simulink library "Braccio_lib"  (R2025b)
settings: Solver=VariableStepAuto  StartTime=0.0  StopTime=10.0  RelTol=1e-3
values from neighbouring files (symbols this model uses):
  dt = 0.01    [Braccio_ini.m]    (also in Braccio_kinematics.m)
  eTol = 0.01    [Braccio_ini.m]
  jnt1 = rigidBodyJoint('jnt1','revolute')    [Braccio_ini.m]    (also in Braccio_kinematics.m)
  jnt2 = rigidBodyJoint('jnt2','revolute')    [Braccio_ini.m]    (also in Braccio_kinematics.m)
  jnt3 = rigidBodyJoint('jnt3','revolute')    [Braccio_ini.m]    (also in Braccio_kinematics.m)
  jnt4 = rigidBodyJoint('jnt4','revolute')    [Braccio_ini.m]    (also in Braccio_kinematics.m)
  jnt5 = rigidBodyJoint('jnt5','revolute')    [Braccio_ini.m]    (also in Braccio_kinematics.m)
undefined symbols (not defined in the file or in its folder): cartesianPath, DiscIntNeverNeededParam, jnt6
libraries: simulink x17, robotcorelib x2
settings Model: Creator=Bender  LastModifiedBy=tom

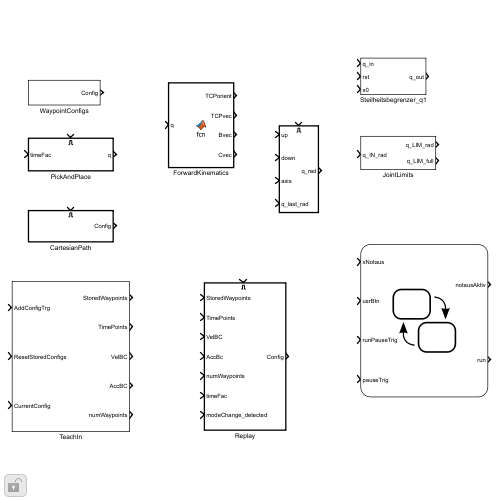
[thumbnail: Simulink's stored preview of the top-level diagram]
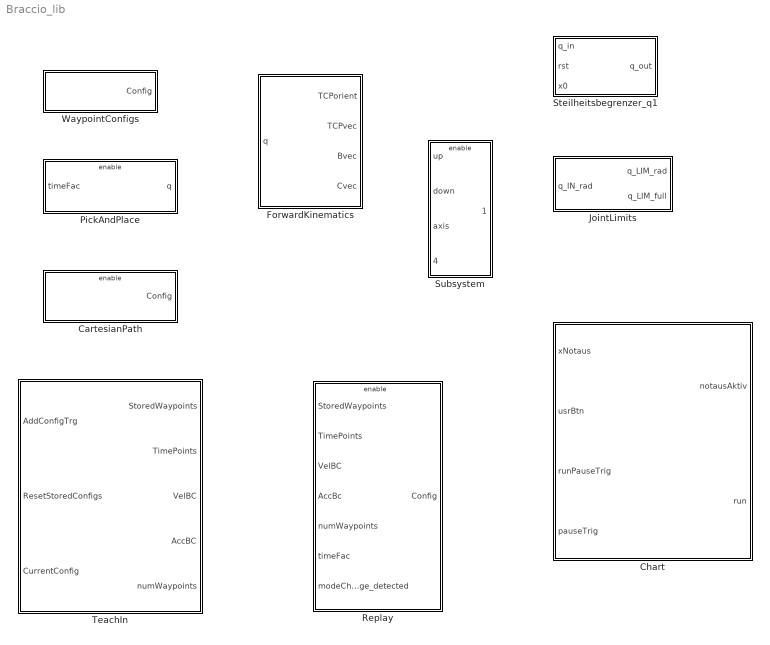
== system Braccio_lib ==
  CartesianPath : Subsystem
  Chart : Stateflow chart  TreatAsAtomicUnit=on
  ForwardKinematics : MATLAB Function  TreatAsAtomicUnit=on
  JointLimits : Subsystem
  PickAndPlace : Subsystem
  Replay : Subsystem
  Steilheitsbegrenzer_q1 : Subsystem
  Subsystem : Subsystem
  TeachIn : Subsystem
  WaypointConfigs : Subsystem

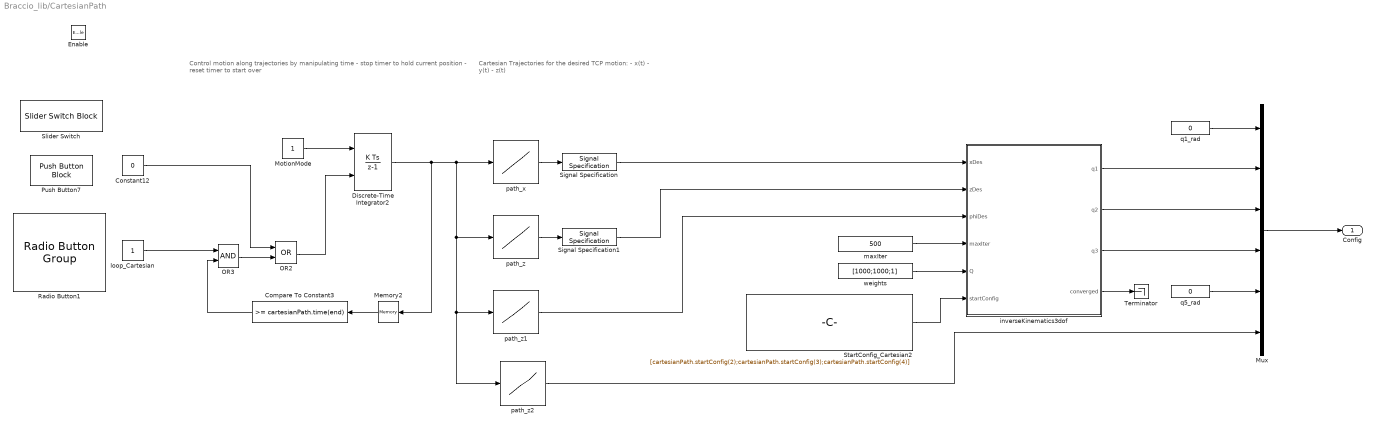
== system Braccio_lib/CartesianPath ==
  note: Cartesian Trajectories for the desired
      | TCP motion:
      | - x(t)
      | - y(t)
      | - z(t)
  note: Control motion along trajectories by manipulating time
      | - stop timer to hold current position
      | - reset timer to start over
  Enable : EnablePort
  Compare To Constant3 : simulink/Logic and Bit Operations/Compare To Constant  relop=>=  const=cartesianPath.time(end)  OutDataTypeStr=boolean
  Constant12 : Constant  Value=0  SampleTime=dt
  Discrete-Time Integrator2 : DiscreteIntegrator  ExternalReset=level  SampleTime=-1  ICPrevOutput=DiscIntNeverNeededParam  ICPrevScaledInput=DiscIntNeverNeededParam
  Memory2 : Memory  InheritSampleTime=on
  MotionMode : Constant  SampleTime=dt
  Mux : Mux  Inputs=6
  OR2 : Logic  Operator=OR  AllPortsSameDT=off  OutDataTypeStr=boolean
  OR3 : Logic  AllPortsSameDT=off  OutDataTypeStr=boolean
  Push Button7 : PushButtonBlock  ButtonText=Reset Time  ButtonType=Latch  IconOnColor=[0.0, 0.39215686274509803, 0.0]  IconOffColor=[0.0, 1.0, 0.0]  OffValue=0.000000
  Radio Button1 : RadioButtonGroup  SelectedLabel=Loop ON  ButtonGroupName=Group
  Signal Specification : SignalSpecification  Dimensions=1
  Signal Specification1 : SignalSpecification  Dimensions=1
  Slider Switch : SliderSwitchBlock
  StartConfig_Cartesian2 : Constant  Value=[cartesianPath.startConfig(2);cartesianPath.startConfig(3);cartesianPath.startConfig(4)]  VectorParams1D=off
  Terminator : Terminator
  inverseKinematics3dof : MATLAB Function  TreatAsAtomicUnit=on
  loop_Cartesian : Constant  SampleTime=dt
  maxIter : Constant  Value=500  SampleTime=dt
  path_x : Lookup_n-D  NumberOfTableDimensions=1  BreakpointsForDimension1=cartesianPath.time  BreakpointsForDimension1DataTypeStr=double  Table=cartesianPath.x  TableDataTypeStr=double  ExtrapMethod=Clip  UseLastTableValue=on  InternalRulePriority=Speed  OutDataTypeStr=double  RndMeth=Simplest
  path_z : Lookup_n-D  NumberOfTableDimensions=1  BreakpointsForDimension1=cartesianPath.time  BreakpointsForDimension1DataTypeStr=double  Table=cartesianPath.z  TableDataTypeStr=double  ExtrapMethod=Clip  UseLastTableValue=on  InternalRulePriority=Speed  OutDataTypeStr=double  RndMeth=Simplest
  path_z1 : Lookup_n-D  NumberOfTableDimensions=1  BreakpointsForDimension1=cartesianPath.time  BreakpointsForDimension1DataTypeStr=double  Table=cartesianPath.angle  TableDataTypeStr=double  ExtrapMethod=Clip  UseLastTableValue=on  InternalRulePriority=Speed  OutDataTypeStr=double  RndMeth=Simplest
  path_z2 : Lookup_n-D  NumberOfTableDimensions=1  BreakpointsForDimension1=cartesianPath.time  BreakpointsForDimension1DataTypeStr=double  Table=cartesianPath.q6  TableDataTypeStr=double  ExtrapMethod=Clip  UseLastTableValue=on  InternalRulePriority=Speed  OutDataTypeStr=double  RndMeth=Simplest
  q1_rad : Constant  Value=0  SampleTime=dt
  q5_rad : Constant  Value=0  SampleTime=dt
  weights : Constant  Value=[1000;1000;1]  VectorParams1D=off  SampleTime=dt
  Config : Outport
  wires:
  Constant12/1 -> OR2/1
  loop_Cartesian/1 -> OR3/1
  OR3/1 -> OR2/2
  Discrete-Time Integrator2/1 -> Memory2/1, path_z2/1, path_z1/1, path_z/1, path_x/1
  OR2/1 -> Discrete-Time Integrator2/2
  Memory2/1 -> Compare To Constant3/1
  Compare To Constant3/1 -> OR3/2
  MotionMode/1 -> Discrete-Time Integrator2/1
  path_x/1 -> Signal Specification/1
  path_z/1 -> Signal Specification1/1
  q1_rad/1 -> Mux/1
  inverseKinematics3dof/1(q1) -> Mux/2
  inverseKinematics3dof/2(q2) -> Mux/3
  inverseKinematics3dof/3(q3) -> Mux/4
  q5_rad/1 -> Mux/5
  path_z2/1 -> Mux/6
  maxIter/1 -> inverseKinematics3dof/4(maxIter)
  weights/1 -> inverseKinematics3dof/5(Q)
  path_z1/1 -> inverseKinematics3dof/3(phiDes)
  Mux/1 -> Config/1
  StartConfig_Cartesian2/1 -> inverseKinematics3dof/6(startConfig)
  inverseKinematics3dof/4(converged) -> Terminator/1
  Signal Specification/1 -> inverseKinematics3dof/1(xDes)
  Signal Specification1/1 -> inverseKinematics3dof/2(zDes)

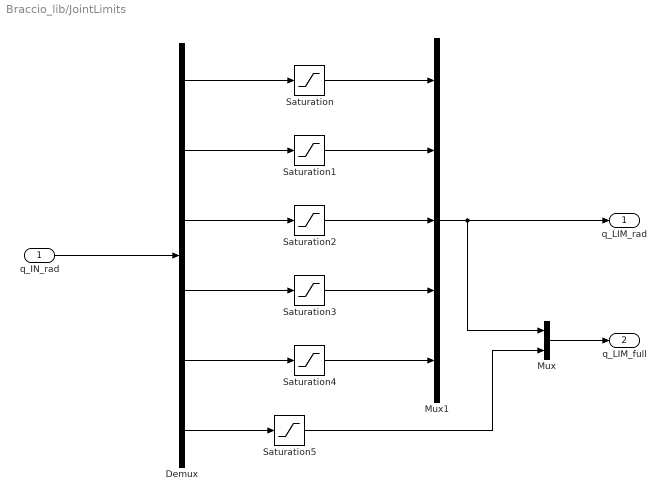
== system Braccio_lib/JointLimits ==
  q_IN_rad : Inport
  Demux : Demux  Outputs=6
  Mux : Mux  Inputs=2
  Mux1 : Mux  Inputs=5
  Saturation : Saturate  UpperLimit=jnt1.PositionLimits(2)  LowerLimit=jnt1.PositionLimits(1)
  Saturation1 : Saturate  UpperLimit=jnt2.PositionLimits(2)  LowerLimit=jnt2.PositionLimits(1)
  Saturation2 : Saturate  UpperLimit=jnt3.PositionLimits(2)  LowerLimit=jnt3.PositionLimits(1)
  Saturation3 : Saturate  UpperLimit=jnt4.PositionLimits(2)  LowerLimit=jnt4.PositionLimits(1)
  Saturation4 : Saturate  UpperLimit=jnt5.PositionLimits(2)  LowerLimit=jnt5.PositionLimits(1)
  Saturation5 : Saturate  UpperLimit=jnt6.PositionLimits(2)  LowerLimit=jnt6.PositionLimits(1)
  q_LIM_rad : Outport
  q_LIM_full : Outport  Port=2
  wires:
  Saturation2/1 -> Mux1/3
  Saturation/1 -> Mux1/1
  Saturation4/1 -> Mux1/5
  Saturation1/1 -> Mux1/2
  Saturation3/1 -> Mux1/4
  Mux1/1 -> Mux/1, q_LIM_rad/1
  q_IN_rad/1 -> Demux/1
  Saturation5/1 -> Mux/2
  Demux/1 -> Saturation/1
  Demux/6 -> Saturation5/1
  Demux/2 -> Saturation1/1
  Demux/3 -> Saturation2/1
  Demux/4 -> Saturation3/1
  Demux/5 -> Saturation4/1
  Mux/1 -> q_LIM_full/1

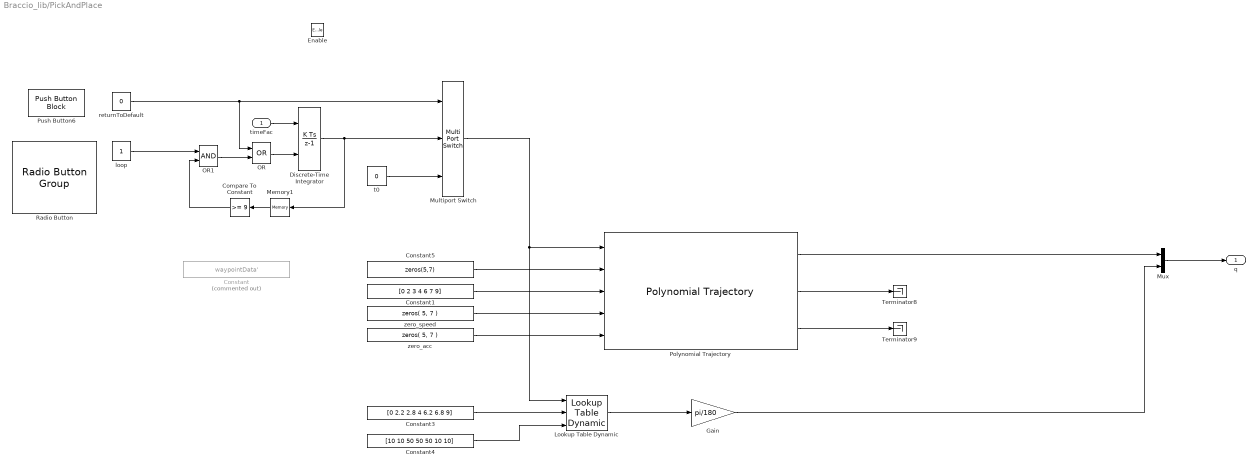
== system Braccio_lib/PickAndPlace ==
  timeFac : Inport
  Enable : EnablePort
  Compare To Constant : simulink/Logic and Bit Operations/Compare To Constant  relop=>=  const=9  OutDataTypeStr=boolean
  Constant : Constant  Commented=on  Value=waypointData'  VectorParams1D=off
  Constant1 : Constant  Value=[0 2 3 4 6 7 9]
  Constant3 : Constant  Value=[0 2.2 2.8 4 6.2 6.8 9]
  Constant4 : Constant  Value=[10 10 50 50 50 10 10]
  Constant5 : Constant  Value=zeros(5,7)  VectorParams1D=off
  Discrete-Time Integrator : DiscreteIntegrator  ExternalReset=level  SampleTime=-1  ICPrevOutput=DiscIntNeverNeededParam  ICPrevScaledInput=DiscIntNeverNeededParam
  Gain : Gain  Gain=pi/180
  Lookup Table Dynamic : simulink/Lookup Tables/Lookup Table Dynamic  LookUpMeth=Interpolation-Use End Values  OutDataType=fixdt('double')  OutScaling=[]  OutputDataTypeScalingMode=Specify via dialog  OutDataTypeStr=double  DoSatur=off
  Memory1 : Memory  InheritSampleTime=on
  Multiport Switch : MultiPortSwitch  DataPortOrder=Zero-based contiguous  Inputs=2  zeroidx=on  SaturateOnIntegerOverflow=off  InputSameDT=off
  Mux : Mux  Inputs=2
  OR : Logic  Operator=OR  AllPortsSameDT=off  OutDataTypeStr=boolean
  OR1 : Logic  AllPortsSameDT=off  OutDataTypeStr=boolean
  Polynomial Trajectory : robotcorelib/Polynomial Trajectory  WaypointSource=External  Waypoints=[ 0, 2, 1, 5, 0; -1, 3, 1, 4, 4 ]  TimePoints=[ 0, 1, 2, 3, 4 ]  TimeInterval=[ 1, 4 ]  Method=Quintic Polynomial  ParameterSource=External  VelocityBoundaryCondition=zeros( 5, 6 )  AccelerationBoundaryCondition=zeros( 5, 6 )  SimulateUsing=Interpreted execution
  Push Button6 : PushButtonBlock  ButtonText=Default Pos  ButtonType=Latch  IconOnColor=[0.0, 0.39215686274509803, 0.0]  IconOffColor=[0.0, 1.0, 0.0]  OffValue=0.000000
  Radio Button : RadioButtonGroup  SelectedLabel=Loop ON  ButtonGroupName=Group
  Terminator8 : Terminator
  Terminator9 : Terminator
  loop : Constant  SampleTime=dt
  returnToDefault : Constant  Value=0  SampleTime=dt
  t0 : Constant  Value=0  SampleTime=dt
  zero_acc : Constant  Value=zeros( 5, 7 )
  zero_speed : Constant  Value=zeros( 5, 7 )
  q : Outport
  wires:
  Gain/1 -> Mux/2
  Constant4/1 -> Lookup Table Dynamic/3
  Constant3/1 -> Lookup Table Dynamic/2
  t0/1 -> Multiport Switch/3
  Discrete-Time Integrator/1 -> Memory1/1, Multiport Switch/2
  Polynomial Trajectory/1 -> Mux/1
  timeFac/1 -> Discrete-Time Integrator/1
  Compare To Constant/1 -> OR1/2
  OR/1 -> Discrete-Time Integrator/2
  Polynomial Trajectory/3 -> Terminator9/1
  Constant1/1 -> Polynomial Trajectory/3
  Memory1/1 -> Compare To Constant/1
  zero_acc/1 -> Polynomial Trajectory/5
  returnToDefault/1 -> OR/1, Multiport Switch/1
  Constant5/1 -> Polynomial Trajectory/2
  zero_speed/1 -> Polynomial Trajectory/4
  loop/1 -> OR1/1
  Polynomial Trajectory/2 -> Terminator8/1
  OR1/1 -> OR/2
  Multiport Switch/1 -> Polynomial Trajectory/1, Lookup Table Dynamic/1
  Mux/1 -> q/1
  Lookup Table Dynamic/1 -> Gain/1

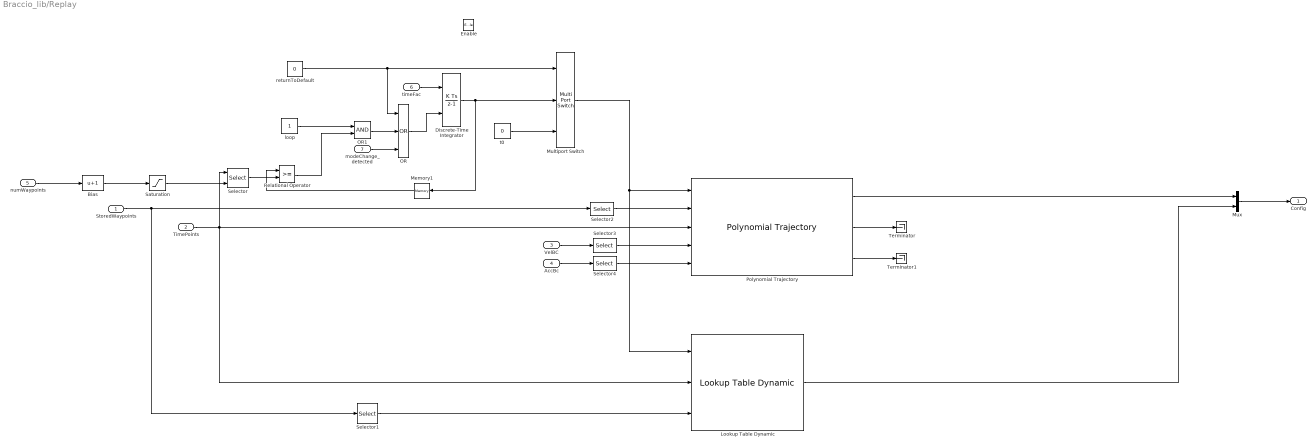
== system Braccio_lib/Replay ==
  StoredWaypoints : Inport
  TimePoints : Inport  Port=2
  VelBC : Inport  Port=3
  AccBc : Inport  Port=4
  numWaypoints : Inport  Port=5
  timeFac : Inport  Port=6
  modeChange_detected : Inport  Port=7
  Enable : EnablePort
  Bias : Bias  Bias=1  SaturateOnIntegerOverflow=off
  Discrete-Time Integrator : DiscreteIntegrator  ExternalReset=level  SampleTime=-1  ICPrevOutput=DiscIntNeverNeededParam  ICPrevScaledInput=DiscIntNeverNeededParam
  Lookup Table Dynamic : simulink/Lookup Tables/Lookup Table Dynamic  LookUpMeth=Interpolation-Use End Values  OutDataType=fixdt('double')  OutScaling=[]  OutputDataTypeScalingMode=Specify via dialog  OutDataTypeStr=double  DoSatur=off
  Memory1 : Memory  InheritSampleTime=on
  Multiport Switch : MultiPortSwitch  DataPortOrder=Zero-based contiguous  Inputs=2  zeroidx=on  SaturateOnIntegerOverflow=off  InputSameDT=off
  Mux : Mux  Inputs=2
  OR : Logic  Operator=OR  Inputs=3  AllPortsSameDT=off  OutDataTypeStr=boolean
  OR1 : Logic  AllPortsSameDT=off  OutDataTypeStr=boolean
  Polynomial Trajectory : robotcorelib/Polynomial Trajectory  WaypointSource=External  Waypoints=[ 0, 2, 1, 5, 0; -1, 3, 1, 4, 4 ]  TimePoints=[ 0, 1, 2, 3, 4 ]  TimeInterval=[ 1, 4 ]  Method=Quintic Polynomial  ParameterSource=External  VelocityBoundaryCondition=zeros( 5, 6 )  AccelerationBoundaryCondition=zeros( 5, 6 )  SimulateUsing=Interpreted execution
  Relational Operator : RelationalOperator  OutDataTypeStr=boolean  RndMeth=Simplest  InputSameDT=off
  Saturation : Saturate  UpperLimit=10  LowerLimit=1
  Selector : Selector  InputPortWidth=10  IndexOptions=Index vector (port)  Indices=[1 3]  OutputSizes=1
  Selector1 : Selector  NumberOfDimensions=2  InputPortWidth=10  IndexOptions=Index vector (dialog),Select all  Indices=6,1  OutputSizes=1,1
  Selector2 : Selector  NumberOfDimensions=2  InputPortWidth=10  IndexOptions=Index vector (dialog),Select all  Indices=[1:5],1  OutputSizes=1,1
  Selector3 : Selector  NumberOfDimensions=2  InputPortWidth=10  IndexOptions=Index vector (dialog),Select all  Indices=[1:5],1  OutputSizes=1,1
  Selector4 : Selector  NumberOfDimensions=2  InputPortWidth=10  IndexOptions=Index vector (dialog),Select all  Indices=[1:5],1  OutputSizes=1,1
  Terminator : Terminator
  Terminator1 : Terminator
  loop : Constant  SampleTime=dt
  returnToDefault : Constant  Value=0  SampleTime=dt
  t0 : Constant  Value=0  SampleTime=dt
  Config : Outport
  wires:
  modeChange_detected/1 -> OR/3
  Polynomial Trajectory/3 -> Terminator1/1
  Polynomial Trajectory/2 -> Terminator/1
  Lookup Table Dynamic/1 -> Mux/2
  OR1/1 -> OR/2
  Multiport Switch/1 -> Lookup Table Dynamic/1, Polynomial Trajectory/1
  Polynomial Trajectory/1 -> Mux/1
  Memory1/1 -> Relational Operator/1
  Mux/1 -> Config/1
  AccBc/1 -> Selector4/1
  returnToDefault/1 -> OR/1, Multiport Switch/1
  loop/1 -> OR1/1
  Relational Operator/1 -> OR1/2
  timeFac/1 -> Discrete-Time Integrator/1
  VelBC/1 -> Selector3/1
  t0/1 -> Multiport Switch/3
  Discrete-Time Integrator/1 -> Memory1/1, Multiport Switch/2
  OR/1 -> Discrete-Time Integrator/2
  Selector1/1 -> Lookup Table Dynamic/3
  TimePoints/1 -> Polynomial Trajectory/3, Lookup Table Dynamic/2, Selector/1
  numWaypoints/1 -> Bias/1
  Selector/1 -> Relational Operator/2
  StoredWaypoints/1 -> Selector1/1, Selector2/1
  Saturation/1 -> Selector/2
  Bias/1 -> Saturation/1
  Selector2/1 -> Polynomial Trajectory/2
  Selector3/1 -> Polynomial Trajectory/4
  Selector4/1 -> Polynomial Trajectory/5

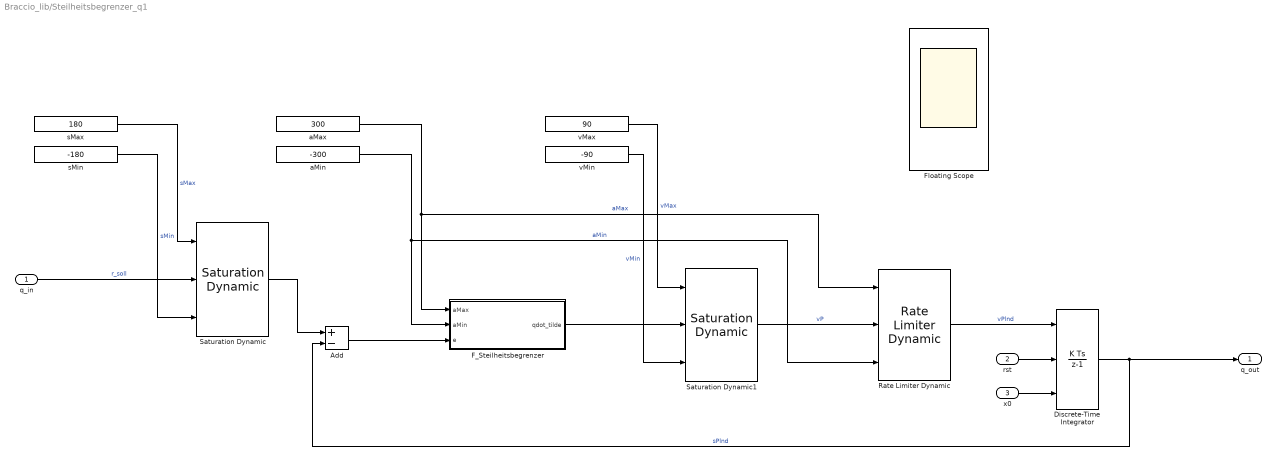
== system Braccio_lib/Steilheitsbegrenzer_q1 ==
  q_in : Inport
  rst : Inport  Port=2
  x0 : Inport  Port=3
  Add : Sum  Inputs=+-
  Discrete-Time Integrator : DiscreteIntegrator  ExternalReset=level  InitialConditionSource=external  SampleTime=-1  ICPrevOutput=DiscIntNeverNeededParam  ICPrevScaledInput=DiscIntNeverNeededParam
  F_Steilheitsbegrenzer : Subsystem
  Floating Scope : Scope
      settings: IsFloating=on  Floating=on  ActiveDisplayYMinimum=-0.27528  ActiveDisplayYMaximum=2.47503  DataLoggingVariableName=ScopeData2
  Rate Limiter Dynamic : simulink/Discontinuities/Rate Limiter Dynamic
  Saturation Dynamic : simulink/Discontinuities/Saturation Dynamic  OutMin=[]  OutMax=[]  OutDataTypeStr=Inherit: Same as second input  OutDataType=fixdt(1, 16)  OutScaling=2^-10  DoSatur=off
  Saturation Dynamic1 : simulink/Discontinuities/Saturation Dynamic  OutMin=[]  OutMax=[]  OutDataTypeStr=Inherit: Same as second input  OutDataType=fixdt(1, 16)  OutScaling=2^-10  DoSatur=off
  aMax : Constant  Value=300  SampleTime=-1
  aMin : Constant  Value=-300  SampleTime=-1
  sMax : Constant  Value=180  SampleTime=-1
  sMin : Constant  Value=-180  SampleTime=-1
  vMax : Constant  Value=90  SampleTime=-1
  vMin : Constant  Value=-90  SampleTime=-1
  q_out : Outport
  wires:
  q_in/1 -> Saturation Dynamic/2  "r_soll"
  aMax/1 -> F_Steilheitsbegrenzer/1(aMax), Rate Limiter Dynamic/1  "aMax"
  Add/1 -> F_Steilheitsbegrenzer/3(e)
  aMin/1 -> F_Steilheitsbegrenzer/2(aMin), Rate Limiter Dynamic/3  "aMin"
  vMin/1 -> Saturation Dynamic1/3  "vMin"
  Saturation Dynamic/1 -> Add/1
  Saturation Dynamic1/1 -> Rate Limiter Dynamic/2  "vP"
  Discrete-Time Integrator/1 -> q_out/1, Add/2  "sPlnd"
  F_Steilheitsbegrenzer/1(qdot_tilde) -> Saturation Dynamic1/2
  sMax/1 -> Saturation Dynamic/1  "sMax"
  rst/1 -> Discrete-Time Integrator/2
  Rate Limiter Dynamic/1 -> Discrete-Time Integrator/1  "vPlnd"
  vMax/1 -> Saturation Dynamic1/1  "vMax"
  sMin/1 -> Saturation Dynamic/3  "sMin"
  x0/1 -> Discrete-Time Integrator/3

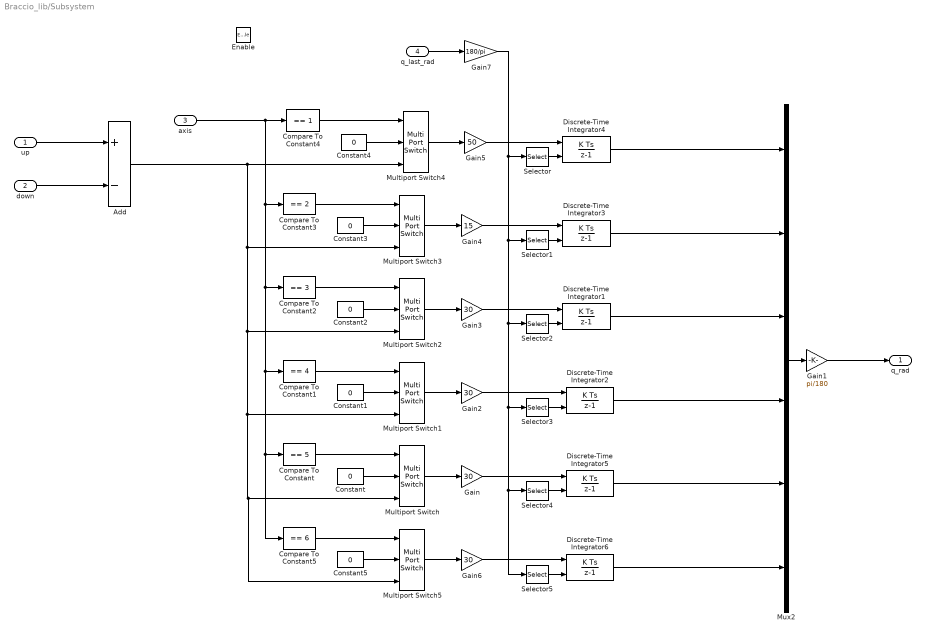
== system Braccio_lib/Subsystem ==
  up : Inport
  down : Inport  Port=2
  axis : Inport  Port=3
  q_last_rad : Inport  Port=4
  Enable : EnablePort  StatesWhenEnabling=reset
  Add : Sum  Inputs=+-
  Compare To Constant : simulink/Logic and Bit Operations/Compare To Constant  relop===  const=5  OutDataTypeStr=boolean
  Compare To Constant1 : simulink/Logic and Bit Operations/Compare To Constant  relop===  const=4  OutDataTypeStr=boolean
  Compare To Constant2 : simulink/Logic and Bit Operations/Compare To Constant  relop===  const=3  OutDataTypeStr=boolean
  Compare To Constant3 : simulink/Logic and Bit Operations/Compare To Constant  relop===  const=2  OutDataTypeStr=boolean
  Compare To Constant4 : simulink/Logic and Bit Operations/Compare To Constant  relop===  const=1  OutDataTypeStr=boolean
  Compare To Constant5 : simulink/Logic and Bit Operations/Compare To Constant  relop===  const=6  OutDataTypeStr=boolean
  Constant{,1..5} (6 alike) : Constant  Value=0  SampleTime=dt
  Discrete-Time Integrator{1,4..6} (4 alike) : DiscreteIntegrator  InitialConditionSource=external  SampleTime=-1  LimitOutput=on  UpperSaturationLimit=90  LowerSaturationLimit=-90  ICPrevOutput=DiscIntNeverNeededParam  ICPrevScaledInput=DiscIntNeverNeededParam
  Discrete-Time Integrator2 : DiscreteIntegrator  InitialConditionSource=external  SampleTime=-1  LimitOutput=on  UpperSaturationLimit=180  LowerSaturationLimit=0  ICPrevOutput=DiscIntNeverNeededParam  ICPrevScaledInput=DiscIntNeverNeededParam
  Discrete-Time Integrator3 : DiscreteIntegrator  InitialConditionSource=external  SampleTime=-1  LimitOutput=on  UpperSaturationLimit=180  LowerSaturationLimit=0  ICPrevOutput=DiscIntNeverNeededParam  ICPrevScaledInput=DiscIntNeverNeededParam
  Gain{,2..3,6} (4 alike) : Gain  Gain=30
  Gain1 : Gain  Gain=pi/180
  Gain4 : Gain  Gain=15
  Gain5 : Gain  Gain=50
  Gain7 : Gain  Gain=180/pi
  Multiport Switch{,1..5} (6 alike) : MultiPortSwitch  DataPortOrder=Zero-based contiguous  Inputs=2  zeroidx=on  SaturateOnIntegerOverflow=off  InputSameDT=off
  Mux2 : Mux  Inputs=6
  Selector : Selector  InputPortWidth=6  IndexOptions=Index vector (dialog)  Indices=1  OutputSizes=1
  Selector1 : Selector  InputPortWidth=6  IndexOptions=Index vector (dialog)  Indices=2  OutputSizes=1
  Selector2 : Selector  InputPortWidth=6  IndexOptions=Index vector (dialog)  Indices=3  OutputSizes=1
  Selector3 : Selector  InputPortWidth=6  IndexOptions=Index vector (dialog)  Indices=4  OutputSizes=1
  Selector4 : Selector  InputPortWidth=6  IndexOptions=Index vector (dialog)  Indices=5  OutputSizes=1
  Selector5 : Selector  InputPortWidth=6  IndexOptions=Index vector (dialog)  Indices=6  OutputSizes=1
  q_rad : Outport  InitialOutput=[0;90;0;90;0;20]*pi/180
  wires:
  Gain7/1 -> Selector/1, Selector1/1, Selector2/1, Selector3/1, Selector4/1, Selector5/1
  Selector5/1 -> Discrete-Time Integrator6/2
  Selector4/1 -> Discrete-Time Integrator5/2
  Selector3/1 -> Discrete-Time Integrator2/2
  Selector2/1 -> Discrete-Time Integrator1/2
  Selector1/1 -> Discrete-Time Integrator3/2
  q_last_rad/1 -> Gain7/1
  Selector/1 -> Discrete-Time Integrator4/2
  Compare To Constant5/1 -> Multiport Switch5/1
  Gain6/1 -> Discrete-Time Integrator6/1
  Multiport Switch5/1 -> Gain6/1
  Constant5/1 -> Multiport Switch5/2
  Add/1 -> Multiport Switch/3, Multiport Switch5/3, Multiport Switch1/3, Multiport Switch2/3, Multiport Switch3/3, Multiport Switch4/3
  Compare To Constant4/1 -> Multiport Switch4/1
  Constant4/1 -> Multiport Switch4/2
  Multiport Switch4/1 -> Gain5/1
  Gain5/1 -> Discrete-Time Integrator4/1
  Gain4/1 -> Discrete-Time Integrator3/1
  Multiport Switch3/1 -> Gain4/1
  Constant3/1 -> Multiport Switch3/2
  Compare To Constant3/1 -> Multiport Switch3/1
  Compare To Constant2/1 -> Multiport Switch2/1
  Constant2/1 -> Multiport Switch2/2
  Multiport Switch2/1 -> Gain3/1
  Gain3/1 -> Discrete-Time Integrator1/1
  Gain2/1 -> Discrete-Time Integrator2/1
  Multiport Switch1/1 -> Gain2/1
  Constant1/1 -> Multiport Switch1/2
  Compare To Constant1/1 -> Multiport Switch1/1
  axis/1 -> Compare To Constant3/1, Compare To Constant/1, Compare To Constant5/1, Compare To Constant1/1, Compare To Constant2/1, Compare To Constant4/1
  Compare To Constant/1 -> Multiport Switch/1
  Constant/1 -> Multiport Switch/2
  up/1 -> Add/1
  Multiport Switch/1 -> Gain/1
  down/1 -> Add/2
  Discrete-Time Integrator6/1 -> Mux2/6
  Mux2/1 -> Gain1/1
  Discrete-Time Integrator5/1 -> Mux2/5
  Discrete-Time Integrator3/1 -> Mux2/2
  Discrete-Time Integrator4/1 -> Mux2/1
  Discrete-Time Integrator1/1 -> Mux2/3
  Discrete-Time Integrator2/1 -> Mux2/4
  Gain/1 -> Discrete-Time Integrator5/1
  Gain1/1 -> q_rad/1

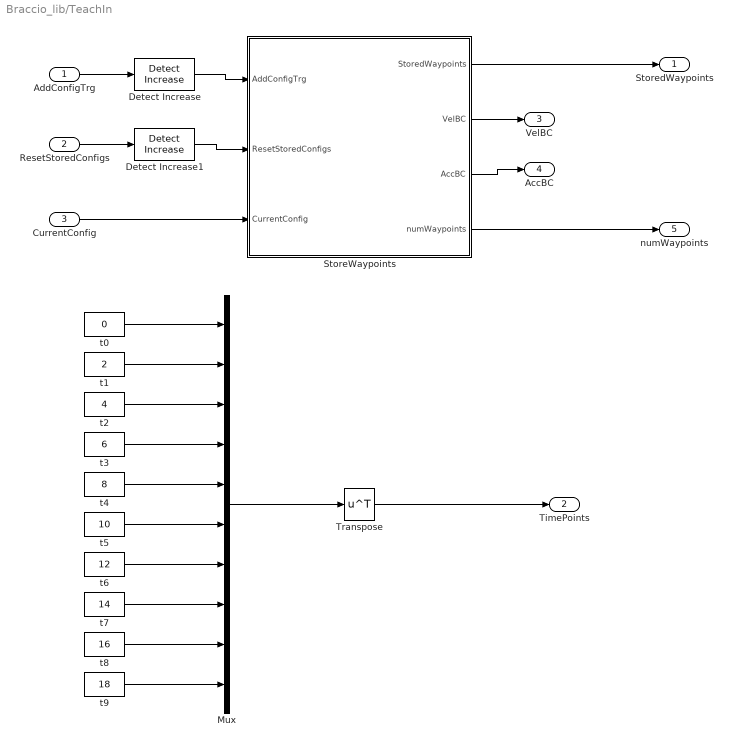
== system Braccio_lib/TeachIn ==
  AddConfigTrg : Inport
  ResetStoredConfigs : Inport  Port=2
  CurrentConfig : Inport  Port=3
  Detect Increase : simulink/Logic and Bit Operations/Detect Increase  vinit=0.0  OutDataTypeStr=boolean
  Detect Increase1 : simulink/Logic and Bit Operations/Detect Increase  vinit=0.0  OutDataTypeStr=boolean
  Mux : Mux  Inputs=10
  StoreWaypoints : MATLAB Function  TreatAsAtomicUnit=on
  Transpose : Math  Operator=transpose
  t0 : Constant  Value=0  SampleTime=dt
  t1 : Constant  Value=2  SampleTime=dt
  t2 : Constant  Value=4  SampleTime=dt
  t3 : Constant  Value=6  SampleTime=dt
  t4 : Constant  Value=8  SampleTime=dt
  t5 : Constant  Value=10  SampleTime=dt
  t6 : Constant  Value=12  SampleTime=dt
  t7 : Constant  Value=14  SampleTime=dt
  t8 : Constant  Value=16  SampleTime=dt
  t9 : Constant  Value=18  SampleTime=dt
  StoredWaypoints : Outport
  TimePoints : Outport  Port=2
  VelBC : Outport  Port=3
  AccBC : Outport  Port=4
  numWaypoints : Outport  Port=5
  wires:
  StoreWaypoints/1(StoredWaypoints) -> StoredWaypoints/1
  Mux/1 -> Transpose/1
  AddConfigTrg/1 -> Detect Increase/1
  ResetStoredConfigs/1 -> Detect Increase1/1
  CurrentConfig/1 -> StoreWaypoints/3(CurrentConfig)
  t0/1 -> Mux/1
  t1/1 -> Mux/2
  t2/1 -> Mux/3
  t4/1 -> Mux/5
  t3/1 -> Mux/4
  t7/1 -> Mux/8
  t8/1 -> Mux/9
  t6/1 -> Mux/7
  t5/1 -> Mux/6
  t9/1 -> Mux/10
  StoreWaypoints/4(numWaypoints) -> numWaypoints/1
  StoreWaypoints/2(VelBC) -> VelBC/1
  StoreWaypoints/3(AccBC) -> AccBC/1
  Transpose/1 -> TimePoints/1
  Detect Increase/1 -> StoreWaypoints/1(AddConfigTrg)
  Detect Increase1/1 -> StoreWaypoints/2(ResetStoredConfigs)

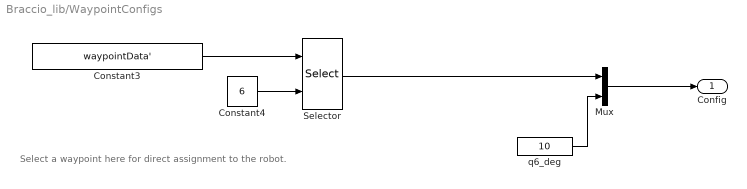
== system Braccio_lib/WaypointConfigs ==
  note: Select a waypoint here for direct assignment to the robot.
  Constant3 : Constant  Value=waypointData'  VectorParams1D=off
  Constant4 : Constant  Value=6
  Mux : Mux  Inputs=2
  Selector : Selector  NumberOfDimensions=2  InputPortWidth=3  IndexOptions=Index vector (dialog),Index vector (port)  Indices=[1:5],1  OutputSizes=1,1
  q6_deg : Constant  Value=10  SampleTime=0.01
  Config : Outport
  wires:
  Constant3/1 -> Selector/1
  Selector/1 -> Mux/1
  Constant4/1 -> Selector/2
  q6_deg/1 -> Mux/2
  Mux/1 -> Config/1

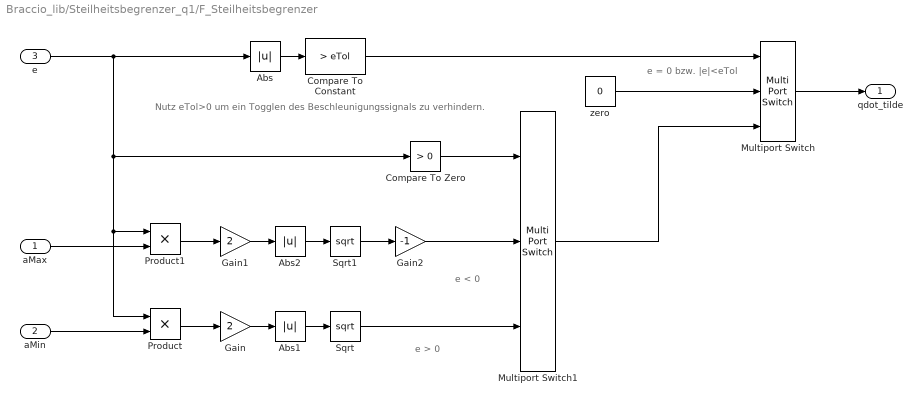
== system Braccio_lib/Steilheitsbegrenzer_q1/F_Steilheitsbegrenzer ==
  note: Nutz eTol>0 um ein Togglen des Beschleunigungssignals zu verhindern.
  note: e < 0
  note: e > 0
  note: e = 0 bzw. |e|<eTol
  aMax : Inport
  aMin : Inport  Port=2
  e : Inport  Port=3
  Abs : Abs  SaturateOnIntegerOverflow=off
  Abs1 : Abs  SaturateOnIntegerOverflow=off
  Abs2 : Abs  SaturateOnIntegerOverflow=off
  Compare To Constant : simulink/Logic and Bit Operations/Compare To Constant  relop=>  const=eTol  OutDataTypeStr=boolean
  Compare To Zero : simulink/Logic and Bit Operations/Compare To Zero  relop=>  OutDataTypeStr=boolean
  Gain : Gain  Gain=2
  Gain1 : Gain  Gain=2
  Gain2 : Gain  Gain=-1
  Multiport Switch : MultiPortSwitch  DataPortOrder=Zero-based contiguous  Inputs=2  zeroidx=on  SaturateOnIntegerOverflow=off  InputSameDT=off
  Multiport Switch1 : MultiPortSwitch  DataPortOrder=Zero-based contiguous  Inputs=2  zeroidx=on  SaturateOnIntegerOverflow=off  InputSameDT=off
  Product : Product
  Product1 : Product
  Sqrt : Sqrt
  Sqrt1 : Sqrt
  zero : Constant  Value=0  SampleTime=-1
  qdot_tilde : Outport
  wires:
  Abs2/1 -> Sqrt1/1
  e/1 -> Abs/1, Product/1, Product1/1, Compare To Zero/1
  zero/1 -> Multiport Switch/2
  Product1/1 -> Gain1/1
  Sqrt1/1 -> Gain2/1
  Multiport Switch1/1 -> Multiport Switch/3
  Abs/1 -> Compare To Constant/1
  Compare To Constant/1 -> Multiport Switch/1
  aMin/1 -> Product/2
  Product/1 -> Gain/1
  Abs1/1 -> Sqrt/1
  Compare To Zero/1 -> Multiport Switch1/1
  Gain1/1 -> Abs2/1
  Sqrt/1 -> Multiport Switch1/3
  Gain/1 -> Abs1/1
  aMax/1 -> Product1/2
  Multiport Switch/1 -> qdot_tilde/1
  Gain2/1 -> Multiport Switch1/2

== matlab function Braccio_lib/TeachIn/StoreWaypoints ==
  data: AddConfigTrg input; StoredWaypoints output size=[6,10]; VelBC output size=[6,10]; AccBC output size=[6,10]; ResetStoredConfigs input; CurrentConfig input; numWaypoints output
function [StoredWaypoints, VelBC, AccBC, numWaypoints]  = fcn(AddConfigTrg,ResetStoredConfigs,CurrentConfig)

persistent WaypointMatrix
persistent VelBCMatrix
persistent AccBCMatrix
persistent columnCounter
persistent startConfig

if isempty(WaypointMatrix) || ResetStoredConfigs
    WaypointMatrix = zeros(6,10);
    columnCounter = 0;
    VelBCMatrix = zeros(6,10);
    AccBCMatrix = zeros(6,10);
    startConfig = zeros(6,1);
end

if AddConfigTrg
    if columnCounter < 9
        columnCounter = columnCounter + 1;
    end
    WaypointMatrix(:,columnCounter) = CurrentConfig;
    if columnCounter==1
        startConfig = CurrentConfig;
    end
    WaypointMatrix(:,columnCounter+1) = startConfig;
    
end

numWaypoints = columnCounter;
StoredWaypoints = WaypointMatrix;
VelBC = VelBCMatrix;
AccBC = AccBCMatrix;

end

== matlab function Braccio_lib/ForwardKinematics ==
  data: TCPorient output; q input; TCPvec output; Bvec output; Cvec output; braccio parameter
function [TCPorient,TCPvec,Bvec,Cvec] = fcn(q, braccio)

q1 = q(1);
q2 = q(2);%braccio.theta2;
q3 = q(3);
q4 = q(4);%braccio.theta4;
q5 = q(5);

% T1
T1 = [cos(q1) -sin(q1)*cos(braccio.alpha1)  sin(q1)*sin(braccio.alpha1)  braccio.a1*cos(q1);
      sin(q1)  cos(q1)*cos(braccio.alpha1) -cos(q1)*sin(braccio.alpha1)  braccio.a1*sin(q1);
      0        sin(braccio.alpha1)          cos(braccio.alpha1)          braccio.d1;
      0        0                            0                            1];

% T2
T2 = [cos(q2) -sin(q2)*cos(braccio.alpha2)  sin(q2)*sin(braccio.alpha2)  braccio.a2*cos(q2);
      sin(q2)  cos(q2)*cos(braccio.alpha2) -cos(q2)*sin(braccio.alpha2)  braccio.a2*sin(q2);
      0        sin(braccio.alpha2)          cos(braccio.alpha2)          braccio.d2;
      0        0                            0                            1];

% T3
T3 = [cos(q3) -sin(q3)*cos(braccio.alpha3)  sin(q3)*sin(braccio.alpha3)  braccio.a3*cos(q3);
      sin(q3)  cos(q3)*cos(braccio.alpha3) -cos(q3)*sin(braccio.alpha3)  braccio.a3*sin(q3);
      0        sin(braccio.alpha3)          cos(braccio.alpha3)          braccio.d3;
      0        0                            0                            1];

% T4
T4 = [cos(q4) -sin(q4)*cos(braccio.alpha4)  sin(q4)*sin(braccio.alpha4)  braccio.a4*cos(q4);
      sin(q4)  cos(q4)*cos(braccio.alpha4) -cos(q4)*sin(braccio.alpha4)  braccio.a4*sin(q4);
      0        sin(braccio.alpha4)          cos(braccio.alpha4)          braccio.d4;
      0        0                            0                            1];

% T5
T5 = [cos(q5) -sin(q5)*cos(braccio.alpha5)  sin(q5)*sin(braccio.alpha5)  (braccio.a5-0.006)*cos(q5);
      sin(q5)  cos(q5)*cos(braccio.alpha5) -cos(q5)*sin(braccio.alpha5)  (braccio.a5-0.006)*sin(q5);
      0        sin(braccio.alpha5)          cos(braccio.alpha5)          braccio.d5+0.05;
      0        0                            0                            1];

%% ----------- TODO --------------------------------------

T15 = T1 * T2 * T3 * T4 * T5;
TCP_hom = T15 * [0; 0; 0; 1]
TCPvec = TCP_hom(1:3);
TCPorient1 = T15(1:3,1:3);
TCPorient = rotm2eul(TCPorient1,'XYZ');

xTCP = TCPvec(1);
yTCP = TCPvec(2);
zTCP = TCPvec(3);

Bvec_hom = T1 * T2 * [0; 0; 0; 1];
Bvec = Bvec_hom(1:3);
Cvec_hom = T1 * T2 * T3 * [0; 0; 0; 1];
Cvec = Cvec_hom(1:3);

== stateflow chart Braccio_lib/Chart ==
  state Pause
    notausAktiv = false;
    run = false;
  state Run
    notausAktiv = false;
    run = true;
  state Notaus
    notausAktiv = true;
    run = false;
  (default) -> Pause
  Pause -> Run [order 2] : [runPauseTrig]
  Run -> Pause [order 2] : [runPauseTrig || pauseTrig]
  Notaus -> Pause : [xNotaus==0 && usrBtn==1]
  Pause -> Notaus [order 1] : [xNotaus==1]
  Run -> Notaus [order 1] : [xNotaus==1]
  data: xNotaus input; notausAktiv output; usrBtn input; runPauseTrig input boolean size=1; run output; pauseTrig input

== matlab function Braccio_lib/CartesianPath/inverseKinematics3dof ==
  data: xDes input; q1 output; q2 output; q3 output; zDes input; phiDes input; maxIter input double size=1; Q input size=[3,1]; converged output; startConfig input
function [q1, q2, q3, converged] = fcn(xDes, zDes, phiDes, maxIter, Q,startConfig)
%#codegen
% INVERSE KINEMATIK FÜR 3-DOF PLANAR-ROBOTER (MIT SCHRITTBETRAGSBEGRENZUNG)

%% 1. KINEMATIK- UND GELENKPARAMETER
l1 = 0.125;   % [m]
l2 = 0.125;   % [m]
l3 = 0.185;   % [m]
a  = 0.0715;  % [m]

q_min = [  15; -135; -180] * (pi/180);
q_max = [ 165;  135;  180] * (pi/180);

%% 2. PERSISTENTER ZUSTAND
persistent qPrev
if isempty(qPrev)
    % Exakter Match für x = 0.365m, z = 0.03m, phi = 0 rad
    qPrev = startConfig;
end

target = [xDes; zDes; phiDes];
q = qPrev; 
tol = 1e-6;
converged = false;
lambda = 1e-2; % Stabilisierte Dämpfung

%% 3. LEVENBERG-MARQUARDT MIT BRANCH-JUMP-SCHUTZ
[cost, g, J, ~] = computeCostAndGradient(q, target, a, l1, l2, l3, Q);
W = diag(Q);

% Maximal zulässige Winkeländerung pro Iterationsschritt (ca. 2.87°)
maxStepRad = 0.05; 

for k = 1:maxIter
    if cost < tol
        converged = true;
        break;
    end
    
    % Gedämpfte Suchrichtung
    H = J' * W * J + lambda * eye(3);
    dq = H \ g;
    
    % Schrittbegrenzung gegen Umklappen in sekundäre Minima
    dqMax = max(abs(dq));
    if dqMax > maxStepRad
        dq = dq * (maxStepRad / dqMax);
    end
    
    step = 1.0;
    accepted = false;
    
    for trial = 1:8
        qTry = max(min(q - step * dq, q_max), q_min);
        [tryCost, tryG, tryJ, ~] = computeCostAndGradient(qTry, target, a, l1, l2, l3, Q);
        
        if tryCost < cost
            q = qTry;
            cost = tryCost;
            g = tryG;
            J = tryJ;
            accepted = true;
            break;
        end
        step = step * 0.5;
    end
    
    if ~accepted
        break;
    end
end

%% 4. ZUSTANDS- UND AUSGABE-UPDATE
qPrev = q;
q1 = q(1);
q2 = q(2);
q3 = q(3);

end

%% HILFSFUNKTION: VORWÄRTSKINEMATIK UND JACOBI
function [cost, g, J, err] = computeCostAndGradient(q, target, a, l1, l2, l3, Q)
c1  = cos(q(1)); 
s1  = sin(q(1)); 
c12 = cos(q(1) + q(2)); 
s12 = sin(q(1) + q(2)); 

q123 = q(1) + q(2) + q(3);
s123 = sin(q123);
c123 = cos(q123);

% Vorwärtskinematik (Matching CAD / IK-Block)
pos = [l1*c1 + l2*c12 + l3*s123;
       a + l1*s1 + l2*s12 - l3*c123;
       q123 - pi/2];

err = pos - target;

% Geometrische Jacobi-Matrix (3x3)
J = [ -l1*s1 - l2*s12 + l3*c123,  -l2*s12 + l3*c123,   l3*c123;
       l1*c1 + l2*c12 + l3*s123,   l2*c12 + l3*s123,   l3*s123;
       1.0,                        1.0,                1.0];

W = diag(Q);
cost = 0.5 * (err' * W * err);
g = J' * (W * err);

end
